simulink model "generic_src"  (Simulink 10.3)
settings: Solver=ode45  StartTime=0.0  StopTime=inf  RelTol=1e-3  EnableMultiTasking=on
undefined symbols (not defined in the file or in its folder): Area_Front, Area_Rear, ay_max_off, ay_max_on, ay_per_mu_max_off, ay_per_mu_max_on, Brake_ratio, brake_valve_ctrl_kP, cat1mode1_higher, cat1mode1_lower, cat1mode2_higher, cat1mode2_lower, cat1mode3_higher, cat1mode3_lower, cat2mode1_higher, cat2mode1_lower, cat2mode2_higher, cat2mode2_lower, cat2mode3_higher, cat2mode3_lower, delta_vel, diff_lock_fac, diff_lock_off, diff_lock_on, ESP_ctrl_kD, ESP_ctrl_kI, ESP_ctrl_kP, ESP_ctrl_restore_kI, ESP_min_throttle_fac, f_ax, f_slip, g, higherlimit_highvel, higherlimit_lowvel, highervel_fac, highervelocity_fac, InitialConditionForIntegrator, limit_acc, limit_selectlow, limit_starting, limit_vdiff, locktime_throttle, lowerlimit_highvel, lowerlimit_lowvel, lowervel_fac, lowervelocity_fac, min_throttle, MPS2KMPH, MSR_ctrl_kD, MSR_ctrl_kI, MSR_ctrl_kP, MSR_min_throttle_fac, PID_kP_sideslip, PID_kP_yawrate, RADpS2RpM, rBrake, RpM2RADpS, SH_SL_switch, sideslip_vel_corr, sidesplip_deviation_max ... (+35)
libraries: CarMaker4SL x136, simulink x55, simulink_extras x6
(part 4 of 9)

== system generic_src/CarMaker/IPG Vehicle/CarAndTrailer/Forces/Tires/TireFR ==
  note: Insert your tire model here.
  Sync_In : Inport
  Load : Inport  Port=2
  vxtrans : Inport  Port=3
  vytrans : Inport  Port=4
  Rim_rotv : Inport  Port=5
  Rim_turnv : Inport  Port=6
  InclinAngle : Inport  Port=7
  muRoad : Inport  Port=8
  Ground{1..11} (11 alike) : Ground
  Terminator{,1..6,12} (8 alike) : Terminator
  Slp : Outport  VectorParamsAs1DForOutWhenUnconnected=off
  Alpha : Outport  Port=2  VectorParamsAs1DForOutWhenUnconnected=off
  TurnSlp : Outport  Port=3  VectorParamsAs1DForOutWhenUnconnected=off
  rBelt_eff : Outport  Port=4  VectorParamsAs1DForOutWhenUnconnected=off
  vBelt : Outport  Port=5  VectorParamsAs1DForOutWhenUnconnected=off
  LongFrc : Outport  Port=6  VectorParamsAs1DForOutWhenUnconnected=off
  SideFrc : Outport  Port=7  VectorParamsAs1DForOutWhenUnconnected=off
  LoadFrc : Outport  Port=8  VectorParamsAs1DForOutWhenUnconnected=off
  OverturnTrq : Outport  Port=9  VectorParamsAs1DForOutWhenUnconnected=off
  RollResist : Outport  Port=10  VectorParamsAs1DForOutWhenUnconnected=off
  AlignTrq : Outport  Port=11  VectorParamsAs1DForOutWhenUnconnected=off
  wires:
  Ground11/1 -> vBelt/1
  Ground10/1 -> rBelt_eff/1
  Ground9/1 -> TurnSlp/1
  Rim_turnv/1 -> Terminator6/1
  Sync_In/1 -> Terminator12/1
  Ground2/1 -> Alpha/1
  Ground3/1 -> LongFrc/1
  Ground4/1 -> SideFrc/1
  Ground5/1 -> OverturnTrq/1
  vxtrans/1 -> Terminator1/1
  vytrans/1 -> Terminator2/1
  Rim_rotv/1 -> Terminator3/1
  InclinAngle/1 -> Terminator4/1
  muRoad/1 -> Terminator5/1
  Load/1 -> Terminator/1
  Ground1/1 -> Slp/1
  Ground6/1 -> LoadFrc/1
  Ground7/1 -> RollResist/1
  Ground8/1 -> AlignTrq/1

== system generic_src/CarMaker/IPG Vehicle/CarAndTrailer/Forces/Tires/TireRL ==
  note: Insert your tire model here.
  Sync_In : Inport
  Load : Inport  Port=2
  vxtrans : Inport  Port=3
  vytrans : Inport  Port=4
  Rim_rotv : Inport  Port=5
  Rim_turnv : Inport  Port=6
  InclinAngle : Inport  Port=7
  muRoad : Inport  Port=8
  Ground{1..11} (11 alike) : Ground
  Terminator{,1..6,12} (8 alike) : Terminator
  Slp : Outport  VectorParamsAs1DForOutWhenUnconnected=off
  Alpha : Outport  Port=2  VectorParamsAs1DForOutWhenUnconnected=off
  TurnSlp : Outport  Port=3  VectorParamsAs1DForOutWhenUnconnected=off
  rBelt_eff : Outport  Port=4  VectorParamsAs1DForOutWhenUnconnected=off
  vBelt : Outport  Port=5  VectorParamsAs1DForOutWhenUnconnected=off
  LongFrc : Outport  Port=6  VectorParamsAs1DForOutWhenUnconnected=off
  SideFrc : Outport  Port=7  VectorParamsAs1DForOutWhenUnconnected=off
  LoadFrc : Outport  Port=8  VectorParamsAs1DForOutWhenUnconnected=off
  OverturnTrq : Outport  Port=9  VectorParamsAs1DForOutWhenUnconnected=off
  RollResist : Outport  Port=10  VectorParamsAs1DForOutWhenUnconnected=off
  AlignTrq : Outport  Port=11  VectorParamsAs1DForOutWhenUnconnected=off
  wires:
  Ground11/1 -> vBelt/1
  Ground10/1 -> rBelt_eff/1
  Ground9/1 -> TurnSlp/1
  Rim_turnv/1 -> Terminator6/1
  Sync_In/1 -> Terminator12/1
  Ground2/1 -> Alpha/1
  Ground3/1 -> LongFrc/1
  Ground4/1 -> SideFrc/1
  Ground5/1 -> OverturnTrq/1
  vxtrans/1 -> Terminator1/1
  vytrans/1 -> Terminator2/1
  Rim_rotv/1 -> Terminator3/1
  InclinAngle/1 -> Terminator4/1
  muRoad/1 -> Terminator5/1
  Load/1 -> Terminator/1
  Ground1/1 -> Slp/1
  Ground6/1 -> LoadFrc/1
  Ground7/1 -> RollResist/1
  Ground8/1 -> AlignTrq/1

== system generic_src/CarMaker/IPG Vehicle/CarAndTrailer/Forces/Tires/TireRR ==
  note: Insert your tire model here.
  Sync_In : Inport
  Load : Inport  Port=2
  vxtrans : Inport  Port=3
  vytrans : Inport  Port=4
  Rim_rotv : Inport  Port=5
  Rim_turnv : Inport  Port=6
  InclinAngle : Inport  Port=7
  muRoad : Inport  Port=8
  Ground{1..11} (11 alike) : Ground
  Terminator{,1..6,12} (8 alike) : Terminator
  Slp : Outport  VectorParamsAs1DForOutWhenUnconnected=off
  Alpha : Outport  Port=2  VectorParamsAs1DForOutWhenUnconnected=off
  TurnSlp : Outport  Port=3  VectorParamsAs1DForOutWhenUnconnected=off
  rBelt_eff : Outport  Port=4  VectorParamsAs1DForOutWhenUnconnected=off
  vBelt : Outport  Port=5  VectorParamsAs1DForOutWhenUnconnected=off
  LongFrc : Outport  Port=6  VectorParamsAs1DForOutWhenUnconnected=off
  SideFrc : Outport  Port=7  VectorParamsAs1DForOutWhenUnconnected=off
  LoadFrc : Outport  Port=8  VectorParamsAs1DForOutWhenUnconnected=off
  OverturnTrq : Outport  Port=9  VectorParamsAs1DForOutWhenUnconnected=off
  RollResist : Outport  Port=10  VectorParamsAs1DForOutWhenUnconnected=off
  AlignTrq : Outport  Port=11  VectorParamsAs1DForOutWhenUnconnected=off
  wires:
  Ground11/1 -> vBelt/1
  Ground10/1 -> rBelt_eff/1
  Ground9/1 -> TurnSlp/1
  Rim_turnv/1 -> Terminator6/1
  Sync_In/1 -> Terminator12/1
  Ground2/1 -> Alpha/1
  Ground3/1 -> LongFrc/1
  Ground4/1 -> SideFrc/1
  Ground5/1 -> OverturnTrq/1
  vxtrans/1 -> Terminator1/1
  vytrans/1 -> Terminator2/1
  Rim_rotv/1 -> Terminator3/1
  InclinAngle/1 -> Terminator4/1
  muRoad/1 -> Terminator5/1
  Load/1 -> Terminator/1
  Ground1/1 -> Slp/1
  Ground6/1 -> LoadFrc/1
  Ground7/1 -> RollResist/1
  Ground8/1 -> AlignTrq/1

== system generic_src/CarMaker/IPG Vehicle/PowerTrain/MCU Example/MyMotorCU/Enabled Subsystem ==
  rotv : Inport
  Trq_trg : Inport  Port=2
  Load : Inport  Port=3
  rotv_trg : Inport  Port=4
  Ratio : Inport  Port=5
  TrqMot_max table : Inport  Port=6
  TrqGen_max table : Inport  Port=7
  rotv_Mot_max : Inport  Port=8
  rotv_Gen_max : Inport  Port=9
  Enable : EnablePort
  Abs : Abs
  Abs1 : Abs
  Abs2 : Abs
  Bus Selector : BusSelector  OutputSignals=x,z
  Bus Selector1 : BusSelector  OutputSignals=x,z
  Compare To Constant : simulink/Logic and Bit Operations/Compare To Constant  relop===  const=-99999  OutDataTypeStr=uint8  ZeroCross=off
  Constant : Constant  Value=0.0
  Constant1 : Constant  Value=0.0
  Gain : Gain  Gain=-1
  Lookup Table Dynamic : simulink/Lookup Tables/Lookup Table Dynamic  LookUpMeth=Interpolation-Use End Values  OutDataType=float('double')  OutScaling=[]  OutputDataTypeScalingMode=Specify via dialog  OutDataTypeStr=float('double')  DoSatur=off
  Lookup Table Dynamic1 : simulink/Lookup Tables/Lookup Table Dynamic  LookUpMeth=Interpolation-Use End Values  OutDataType=float('double')  OutScaling=[]  OutputDataTypeScalingMode=Specify via dialog  OutDataTypeStr=float('double')  DoSatur=off
  MotMode : Subsystem
  Product : Product  RndMeth=Zero
  Product1 : Product  RndMeth=Zero
  Product2 : Product  RndMeth=Zero
  Saturation : Saturate  UpperLimit=1  LowerLimit=-1
  Switch : Switch  Criteria=u2 ~= 0
  Switch1 : Switch  Criteria=u2 ~= 0
  Switch2 : Switch  Criteria=u2 ~= 0
  if condition : Subsystem
  rotv Copy : InportShadow
  Load out : Outport  VectorParamsAs1DForOutWhenUnconnected=off
  TrqMot_max : Outport  Port=2  VectorParamsAs1DForOutWhenUnconnected=off
  TrqGen_max : Outport  Port=3  VectorParamsAs1DForOutWhenUnconnected=off
  wires:
  rotv Copy/1 -> if condition/2(rotv)
  Bus Selector/2 -> Lookup Table Dynamic/3  "<z>"
  Lookup Table Dynamic/1 -> Product1/2
  Abs2/1 -> Switch/1
  Abs1/1 -> Switch/3
  Product/1 -> Lookup Table Dynamic1/1, Lookup Table Dynamic/1  "rotv"
  rotv_trg/1 -> if condition/1(rotv_trg)
  if condition/1(Boolean) -> Switch2/2
  Switch1/1 -> Switch2/3  "Load"
  Constant1/1 -> Switch2/1
  Switch2/1 -> Load out/1
  Saturation/1 -> Switch1/3
  Constant/1 -> Switch1/1
  Compare To Constant/1 -> Switch1/2
  Load/1 -> Saturation/1, Compare To Constant/1
  Trq_trg/1 -> MotMode/1(Trq_trg)
  MotMode/1(Boolean) -> Switch/2
  Gain/1 -> Product2/2
  Product2/1 -> TrqGen_max/1
  Product1/1 -> TrqMot_max/1
  Switch/1 -> if condition/3(lim_rotv)  "lim_rotv"
  rotv_Mot_max/1 -> Abs2/1
  rotv_Gen_max/1 -> Abs1/1
  Lookup Table Dynamic1/1 -> Gain/1
  Bus Selector1/2 -> Lookup Table Dynamic1/3  "<z>"
  Bus Selector1/1 -> Lookup Table Dynamic1/2  "<x>"
  TrqGen_max table/1 -> Bus Selector1/1
  Bus Selector/1 -> Lookup Table Dynamic/2  "<x>"
  TrqMot_max table/1 -> Bus Selector/1
  Abs/1 -> Product/1
  Ratio/1 -> Product1/1, Product2/1, Product/2
  rotv/1 -> MotMode/2(rotv), Abs/1

== system generic_src/CarMaker/IPG Vehicle/PowerTrain/MCU Example/MyMotorCU/ReturnZero ==
  Enable : EnablePort
  Bus Creator : BusCreator  Inputs=3
  Constant : Constant  Value=0.0
  Constant1 : Constant  Value=0.0
  Constant2 : Constant  Value=0.0
  Signal Conversion : SignalConversion  ConversionOutput=Bus copy  OverrideOpt=off
  ReturnZero : Outport  VectorParamsAs1DForOutWhenUnconnected=off
  wires:
  Signal Conversion/1 -> ReturnZero/1
  Constant2/1 -> Bus Creator/3  "TrqGen_max"
  Constant1/1 -> Bus Creator/2  "TrqMot_max"
  Constant/1 -> Bus Creator/1  "Load"
  Bus Creator/1 -> Signal Conversion/1

== system generic_src/CarMaker/IPG Vehicle/PowerTrain/MCU Example/PTMotorCU_In/CreateBus MCU ISGIn ==
  In : Inport
  BusCreator : BusCreator  Inputs=12
  Demux : Demux  Outputs=12
      settings: DisplayOption=none
  Out : Outport  VectorParamsAs1DForOutWhenUnconnected=off
  wires:
  Demux/6 -> BusCreator/6  "MCU ISGIn PwrElec"
  Demux/4 -> BusCreator/4  "MCU ISGIn rotv"
  Demux/3 -> BusCreator/3  "MCU ISGIn rotv_trg"
  Demux/2 -> BusCreator/2  "MCU ISGIn Trq"
  Demux/8 -> BusCreator/8  "MCU ISGIn Current_d"
  Demux/9 -> BusCreator/9  "MCU ISGIn Current_q"
  In/1 -> Demux/1
  Demux/7 -> BusCreator/7  "MCU ISGIn VoltBatt"
  BusCreator/1 -> Out/1
  Demux/1 -> BusCreator/1  "MCU ISGIn Trq_trg"
  Demux/5 -> BusCreator/5  "MCU ISGIn rot"
  Demux/10 -> BusCreator/10  "MCU ISGIn Current_u"
  Demux/11 -> BusCreator/11  "MCU ISGIn Current_v"
  Demux/12 -> BusCreator/12  "MCU ISGIn Current_w"

== system generic_src/CarMaker/IPG Vehicle/PowerTrain/MCU Example/PTMotorCU_In/CreateBus MCU ISGOut ==
  In : Inport
  BusCreator : BusCreator  Inputs=1
  Demux : Demux  Outputs=1
      settings: DisplayOption=none
  Out : Outport  VectorParamsAs1DForOutWhenUnconnected=off
  wires:
  Demux/1 -> BusCreator/1  "MCU ISGIn Load"
  BusCreator/1 -> Out/1
  In/1 -> Demux/1

== system generic_src/CarMaker/IPG Vehicle/PowerTrain/MCU Example/PTMotorCU_In/CreateBus MCU Ignition ==
  In : Inport
  BusCreator : BusCreator  Inputs=1
  Demux : Demux  Outputs=1
      settings: DisplayOption=none
  Out : Outport  VectorParamsAs1DForOutWhenUnconnected=off
  wires:
  Demux/1 -> BusCreator/1  "MCU Ignition"
  BusCreator/1 -> Out/1
  In/1 -> Demux/1

== system generic_src/CarMaker/IPG Vehicle/PowerTrain/MCU Example/PTMotorCU_In/CreateBus MCU MotorIn0 ==
  In : Inport
  BusCreator1 : BusCreator  Inputs=12
  Demux1 : Demux  Outputs=12
      settings: DisplayOption=none
  Out : Outport  VectorParamsAs1DForOutWhenUnconnected=off
  wires:
  In/1 -> Demux1/1
  Demux1/12 -> BusCreator1/12  "MCU MotorIn0 Current_w"
  Demux1/10 -> BusCreator1/10  "MCU MotorIn0 Current_u"
  Demux1/6 -> BusCreator1/6  "MCU MotorIn0 PwrElec"
  Demux1/7 -> BusCreator1/7  "MCU MotorIn0 VoltBatt"
  Demux1/9 -> BusCreator1/9  "MCU MotorIn0 Current_q"
  Demux1/1 -> BusCreator1/1  "MCU MotorIn0 Trq_trg"
  Demux1/3 -> BusCreator1/3  "MCU MotorIn0 rotv_trg"
  BusCreator1/1 -> Out/1
  Demux1/2 -> BusCreator1/2  "MCU MotorIn0 Trq"
  Demux1/4 -> BusCreator1/4  "MCU MotorIn0 rotv"
  Demux1/11 -> BusCreator1/11  "MCU MotorIn0 Current_v"
  Demux1/8 -> BusCreator1/8  "MCU MotorIn0 Current_d"
  Demux1/5 -> BusCreator1/5  "MCU MotorIn0 rot"

== system generic_src/CarMaker/IPG Vehicle/PowerTrain/MCU Example/PTMotorCU_In/CreateBus MCU MotorIn1 ==
  In : Inport
  BusCreator1 : BusCreator  Inputs=12
  Demux1 : Demux  Outputs=12
      settings: DisplayOption=none
  Out : Outport  VectorParamsAs1DForOutWhenUnconnected=off
  wires:
  Demux1/4 -> BusCreator1/4  "MCU MotorIn1 rotv"
  Demux1/10 -> BusCreator1/10  "MCU MotorIn1 Current_u"
  BusCreator1/1 -> Out/1
  Demux1/7 -> BusCreator1/7  "MCU MotorIn1 VoltBatt"
  Demux1/8 -> BusCreator1/8  "MCU MotorIn1 Current_d"
  Demux1/1 -> BusCreator1/1  "MCU MotorIn1 Trq_trg"
  Demux1/9 -> BusCreator1/9  "MCU MotorIn1 Current_q"
  Demux1/5 -> BusCreator1/5  "MCU MotorIn1 rot"
  In/1 -> Demux1/1
  Demux1/2 -> BusCreator1/2  "MCU MotorIn1 Trq"
  Demux1/3 -> BusCreator1/3  "MCU MotorIn1 rotv_trg"
  Demux1/6 -> BusCreator1/6  "MCU MotorIn1 PwrElec"
  Demux1/12 -> BusCreator1/12  "MCU MotorIn1 Current_w"
  Demux1/11 -> BusCreator1/11  "MCU MotorIn1 Current_v"

== system generic_src/CarMaker/IPG Vehicle/PowerTrain/MCU Example/PTMotorCU_In/CreateBus MCU MotorIn2 ==
  In : Inport
  BusCreator1 : BusCreator  Inputs=12
  Demux1 : Demux  Outputs=12
      settings: DisplayOption=none
  Out : Outport  VectorParamsAs1DForOutWhenUnconnected=off
  wires:
  Demux1/1 -> BusCreator1/1  "MCU MotorIn2 Trq_trg"
  Demux1/5 -> BusCreator1/5  "MCU MotorIn2 rot"
  BusCreator1/1 -> Out/1
  Demux1/9 -> BusCreator1/9  "MCU MotorIn2 Current_q"
  Demux1/3 -> BusCreator1/3  "MCU MotorIn2 rotv_trg"
  Demux1/4 -> BusCreator1/4  "MCU MotorIn2 rotv"
  Demux1/7 -> BusCreator1/7  "MCU MotorIn2 VoltBatt"
  Demux1/12 -> BusCreator1/12  "MCU MotorIn2 Current_w"
  In/1 -> Demux1/1
  Demux1/2 -> BusCreator1/2  "MCU MotorIn2 Trq"
  Demux1/8 -> BusCreator1/8  "MCU MotorIn2 Current_d"
  Demux1/11 -> BusCreator1/11  "MCU MotorIn2 Current_v"
  Demux1/6 -> BusCreator1/6  "MCU MotorIn2 PwrElec"
  Demux1/10 -> BusCreator1/10  "MCU MotorIn2 Current_u"

== system generic_src/CarMaker/IPG Vehicle/PowerTrain/MCU Example/PTMotorCU_In/CreateBus MCU MotorIn3 ==
  In : Inport
  BusCreator1 : BusCreator  Inputs=12
  Demux1 : Demux  Outputs=12
      settings: DisplayOption=none
  Out : Outport  VectorParamsAs1DForOutWhenUnconnected=off
  wires:
  BusCreator1/1 -> Out/1
  Demux1/5 -> BusCreator1/5  "MCU MotorIn3 rot"
  Demux1/7 -> BusCreator1/7  "MCU MotorIn3 VoltBatt"
  Demux1/6 -> BusCreator1/6  "MCU MotorIn3 PwrElec"
  Demux1/8 -> BusCreator1/8  "MCU MotorIn3 Current_d"
  Demux1/9 -> BusCreator1/9  "MCU MotorIn3 Current_q"
  Demux1/11 -> BusCreator1/11  "MCU MotorIn3 Current_v"
  Demux1/1 -> BusCreator1/1  "MCU MotorIn3 Trq_trg"
  Demux1/10 -> BusCreator1/10  "MCU MotorIn3 Current_u"
  Demux1/4 -> BusCreator1/4  "MCU MotorIn3 rotv"
  Demux1/12 -> BusCreator1/12  "MCU MotorIn3 Current_w"
  Demux1/2 -> BusCreator1/2  "MCU MotorIn3 Trq"
  In/1 -> Demux1/1
  Demux1/3 -> BusCreator1/3  "MCU MotorIn3 rotv_trg"

== system generic_src/CarMaker/IPG Vehicle/PowerTrain/MCU Example/PTMotorCU_In/CreateBus MCU MotorOut0 ==
  In : Inport
  BusCreator : BusCreator  Inputs=1
  Demux : Demux  Outputs=1
      settings: DisplayOption=none
  Out : Outport  VectorParamsAs1DForOutWhenUnconnected=off
  wires:
  Demux/1 -> BusCreator/1  "MCU MotorOut0 Load"
  BusCreator/1 -> Out/1
  In/1 -> Demux/1

== system generic_src/CarMaker/IPG Vehicle/PowerTrain/MCU Example/PTMotorCU_In/CreateBus MCU MotorOut1 ==
  In : Inport
  BusCreator : BusCreator  Inputs=1
  Demux : Demux  Outputs=1
      settings: DisplayOption=none
  Out : Outport  VectorParamsAs1DForOutWhenUnconnected=off
  wires:
  Demux/1 -> BusCreator/1  "MCU MotorOut1 Load"
  In/1 -> Demux/1
  BusCreator/1 -> Out/1

== system generic_src/CarMaker/IPG Vehicle/PowerTrain/MCU Example/PTMotorCU_In/CreateBus MCU MotorOut2 ==
  In : Inport
  BusCreator : BusCreator  Inputs=1
  Demux : Demux  Outputs=1
      settings: DisplayOption=none
  Out : Outport  VectorParamsAs1DForOutWhenUnconnected=off
  wires:
  Demux/1 -> BusCreator/1  "MCU MotorOut2 Load"
  BusCreator/1 -> Out/1
  In/1 -> Demux/1

== system generic_src/CarMaker/IPG Vehicle/PowerTrain/MCU Example/PTMotorCU_In/CreateBus MCU MotorOut3 ==
  In : Inport
  BusCreator : BusCreator  Inputs=1
  Demux : Demux  Outputs=1
      settings: DisplayOption=none
  Out : Outport  VectorParamsAs1DForOutWhenUnconnected=off
  wires:
  Demux/1 -> BusCreator/1  "MCU MotorOut3 Load"
  BusCreator/1 -> Out/1
  In/1 -> Demux/1

== system generic_src/CarMaker/IPG Vehicle/PowerTrain/MCU Example/PTMotorCU_In/CreateBus MCU_Cfg ISG ==
  In : Inport
  BusCreator : BusCreator  Inputs=8
  Demux : Demux  Outputs=8
      settings: DisplayOption=none
  Out : Outport  VectorParamsAs1DForOutWhenUnconnected=off
  wires:
  BusCreator/1 -> Out/1
  In/1 -> Demux/1
  Demux/4 -> BusCreator/4  "MCU_Cfg ISG rotv_Gen_max"
  Demux/1 -> BusCreator/1  "MCU_Cfg ISG CtrlMode"
  Demux/2 -> BusCreator/2  "MCU_Cfg ISG Ratio"
  Demux/3 -> BusCreator/3  "MCU_Cfg ISG rotv_Mot_max"
  Demux/5 -> BusCreator/5  "MCU_Cfg ISG nPolePairs"
  Demux/6 -> BusCreator/6  "MCU_Cfg ISG L_d"
  Demux/7 -> BusCreator/7  "MCU_Cfg ISG L_q"
  Demux/8 -> BusCreator/8  "MCU_Cfg ISG Psi_PM"

== system generic_src/CarMaker/IPG Vehicle/PowerTrain/MCU Example/PTMotorCU_In/CreateBus MCU_Cfg Misc ==
  In : Inport
  BusCreator : BusCreator  Inputs=1
  Demux : Demux  Outputs=1
      settings: DisplayOption=none
  Out : Outport  VectorParamsAs1DForOutWhenUnconnected=off
  wires:
  Demux/1 -> BusCreator/1  "MCU_Cfg nMotor"
  BusCreator/1 -> Out/1
  In/1 -> Demux/1

== system generic_src/CarMaker/IPG Vehicle/PowerTrain/MCU Example/PTMotorCU_In/CreateBus MCU_Cfg Motor0 ==
  In : Inport
  BusCreator1 : BusCreator  Inputs=8
  Demux1 : Demux  Outputs=8
      settings: DisplayOption=none
  Out : Outport  VectorParamsAs1DForOutWhenUnconnected=off
  wires:
  Demux1/4 -> BusCreator1/4  "MCU_Cfg Motor0 rotv_Gen_max"
  Demux1/2 -> BusCreator1/2  "MCU_Cfg Motor0 Ratio"
  Demux1/3 -> BusCreator1/3  "MCU_Cfg Motor0 rotv_Mot_max"
  Demux1/1 -> BusCreator1/1  "MCU_Cfg Motor0 CtrlMode"
  In/1 -> Demux1/1
  BusCreator1/1 -> Out/1
  Demux1/5 -> BusCreator1/5  "MCU_Cfg Motor0 nPolePairs"
  Demux1/6 -> BusCreator1/6  "MCU_Cfg Motor0 L_d"
  Demux1/7 -> BusCreator1/7  "MCU_Cfg Motor0 L_q"
  Demux1/8 -> BusCreator1/8  "MCU_Cfg Motor0 Psi_PM"

== system generic_src/CarMaker/IPG Vehicle/PowerTrain/MCU Example/PTMotorCU_In/CreateBus MCU_Cfg Motor1 ==
  In : Inport
  BusCreator : BusCreator  Inputs=8
  Demux : Demux  Outputs=8
      settings: DisplayOption=none
  Out : Outport  VectorParamsAs1DForOutWhenUnconnected=off
  wires:
  Demux/4 -> BusCreator/4  "MCU_Cfg Motor1 rotv_Gen_max"
  Demux/2 -> BusCreator/2  "MCU_Cfg Motor1 Ratio"
  Demux/3 -> BusCreator/3  "MCU_Cfg Motor1 rotv_Mot_max"
  Demux/1 -> BusCreator/1  "MCU_Cfg Motor1 CtrlMode"
  In/1 -> Demux/1
  BusCreator/1 -> Out/1
  Demux/5 -> BusCreator/5  "MCU_Cfg Motor1 nPolePairs"
  Demux/6 -> BusCreator/6  "MCU_Cfg Motor1 L_d"
  Demux/7 -> BusCreator/7  "MCU_Cfg Motor1 L_q"
  Demux/8 -> BusCreator/8  "MCU_Cfg Motor1 Psi_PM"

== system generic_src/CarMaker/IPG Vehicle/PowerTrain/MCU Example/PTMotorCU_In/CreateBus MCU_Cfg Motor2 ==
  In : Inport
  BusCreator : BusCreator  Inputs=8
  Demux : Demux  Outputs=8
      settings: DisplayOption=none
  Out : Outport  VectorParamsAs1DForOutWhenUnconnected=off
  wires:
  Demux/4 -> BusCreator/4  "MCU_Cfg Motor2 rotv_Gen_max"
  Demux/1 -> BusCreator/1  "MCU_Cfg Motor2 CtrlMode"
  Demux/2 -> BusCreator/2  "MCU_Cfg Motor2 Ratio"
  Demux/3 -> BusCreator/3  "MCU_Cfg Motor2 rotv_Mot_max"
  BusCreator/1 -> Out/1
  In/1 -> Demux/1
  Demux/5 -> BusCreator/5  "MCU_Cfg Motor2 nPolePairs"
  Demux/6 -> BusCreator/6  "MCU_Cfg Motor2 L_d"
  Demux/7 -> BusCreator/7  "MCU_Cfg Motor2 L_q"
  Demux/8 -> BusCreator/8  "MCU_Cfg Motor2 Psi_PM"

== system generic_src/CarMaker/IPG Vehicle/PowerTrain/MCU Example/PTMotorCU_In/CreateBus MCU_Cfg Motor3 ==
  In : Inport
  BusCreator : BusCreator  Inputs=8
  Demux : Demux  Outputs=8
      settings: DisplayOption=none
  Out : Outport  VectorParamsAs1DForOutWhenUnconnected=off
  wires:
  Demux/4 -> BusCreator/4  "MCU_Cfg Motor3 rotv_Gen_max"
  Demux/1 -> BusCreator/1  "MCU_Cfg Motor3 CtrlMode"
  Demux/2 -> BusCreator/2  "MCU_Cfg Motor3 Ratio"
  Demux/3 -> BusCreator/3  "MCU_Cfg Motor3 rotv_Mot_max"
  BusCreator/1 -> Out/1
  In/1 -> Demux/1
  Demux/5 -> BusCreator/5  "MCU_Cfg Motor3 nPolePairs"
  Demux/6 -> BusCreator/6  "MCU_Cfg Motor3 L_d"
  Demux/7 -> BusCreator/7  "MCU_Cfg Motor3 L_q"
  Demux/8 -> BusCreator/8  "MCU_Cfg Motor3 Psi_PM"

== system generic_src/CarMaker/IPG Vehicle/PowerTrain/PTControl Example/PTC ClutchOut/CreateBus PTC ClutchOut0 ==
  In : Inport
  BusCreator : BusCreator  Inputs=3
  Demux : Demux  Outputs=3
      settings: DisplayOption=none
  Out : Outport  VectorParamsAs1DForOutWhenUnconnected=off
  wires:
  Demux/3 -> BusCreator/3  "PTC ClutchOut0 Trq_out_trg"
  Demux/2 -> BusCreator/2  "PTC ClutchOut0 rotv_out_trg"
  Demux/1 -> BusCreator/1  "PTC ClutchOut0 Pos"
  BusCreator/1 -> Out/1
  In/1 -> Demux/1

== system generic_src/CarMaker/IPG Vehicle/PowerTrain/PTControl Example/PTC ClutchOut/CreateBus PTC ClutchOut1 ==
  In : Inport
  BusCreator : BusCreator  Inputs=3
  Demux : Demux  Outputs=3
      settings: DisplayOption=none
  Out : Outport  VectorParamsAs1DForOutWhenUnconnected=off
  wires:
  Demux/3 -> BusCreator/3  "PTC ClutchOut1 Trq_out_trg"
  Demux/2 -> BusCreator/2  "PTC ClutchOut1 rotv_out_trg"
  Demux/1 -> BusCreator/1  "PTC ClutchOut1 Pos"
  BusCreator/1 -> Out/1
  In/1 -> Demux/1

== system generic_src/CarMaker/IPG Vehicle/PowerTrain/PTControl Example/PTC ClutchOut/CreateBus PTC ClutchOut10 ==
  In : Inport
  BusCreator : BusCreator  Inputs=3
  Demux : Demux  Outputs=3
      settings: DisplayOption=none
  Out : Outport  VectorParamsAs1DForOutWhenUnconnected=off
  wires:
  Demux/3 -> BusCreator/3  "PTC ClutchOut10 Trq_out_trg"
  Demux/2 -> BusCreator/2  "PTC ClutchOut10 rotv_out_trg"
  Demux/1 -> BusCreator/1  "PTC ClutchOut10 Pos"
  BusCreator/1 -> Out/1
  In/1 -> Demux/1

== system generic_src/CarMaker/IPG Vehicle/PowerTrain/PTControl Example/PTC ClutchOut/CreateBus PTC ClutchOut11 ==
  In : Inport
  BusCreator : BusCreator  Inputs=3
  Demux : Demux  Outputs=3
      settings: DisplayOption=none
  Out : Outport  VectorParamsAs1DForOutWhenUnconnected=off
  wires:
  Demux/3 -> BusCreator/3  "PTC ClutchOut11 Trq_out_trg"
  Demux/2 -> BusCreator/2  "PTC ClutchOut11 rotv_out_trg"
  Demux/1 -> BusCreator/1  "PTC ClutchOut11 Pos"
  BusCreator/1 -> Out/1
  In/1 -> Demux/1

== system generic_src/CarMaker/IPG Vehicle/PowerTrain/PTControl Example/PTC ClutchOut/CreateBus PTC ClutchOut2 ==
  In : Inport
  BusCreator : BusCreator  Inputs=3
  Demux : Demux  Outputs=3
      settings: DisplayOption=none
  Out : Outport  VectorParamsAs1DForOutWhenUnconnected=off
  wires:
  Demux/3 -> BusCreator/3  "PTC ClutchOut2 Trq_out_trg"
  Demux/2 -> BusCreator/2  "PTC ClutchOut2 rotv_out_trg"
  Demux/1 -> BusCreator/1  "PTC ClutchOut2 Pos"
  BusCreator/1 -> Out/1
  In/1 -> Demux/1

== system generic_src/CarMaker/IPG Vehicle/PowerTrain/PTControl Example/PTC ClutchOut/CreateBus PTC ClutchOut3 ==
  In : Inport
  BusCreator : BusCreator  Inputs=3
  Demux : Demux  Outputs=3
      settings: DisplayOption=none
  Out : Outport  VectorParamsAs1DForOutWhenUnconnected=off
  wires:
  Demux/3 -> BusCreator/3  "PTC ClutchOut3 Trq_out_trg"
  Demux/2 -> BusCreator/2  "PTC ClutchOut3 rotv_out_trg"
  Demux/1 -> BusCreator/1  "PTC ClutchOut3 Pos"
  BusCreator/1 -> Out/1
  In/1 -> Demux/1

== system generic_src/CarMaker/IPG Vehicle/PowerTrain/PTControl Example/PTC ClutchOut/CreateBus PTC ClutchOut4 ==
  In : Inport
  BusCreator : BusCreator  Inputs=3
  Demux : Demux  Outputs=3
      settings: DisplayOption=none
  Out : Outport  VectorParamsAs1DForOutWhenUnconnected=off
  wires:
  Demux/3 -> BusCreator/3  "PTC ClutchOut4 Trq_out_trg"
  Demux/2 -> BusCreator/2  "PTC ClutchOut4 rotv_out_trg"
  Demux/1 -> BusCreator/1  "PTC ClutchOut4 Pos"
  BusCreator/1 -> Out/1
  In/1 -> Demux/1

== system generic_src/CarMaker/IPG Vehicle/PowerTrain/PTControl Example/PTC ClutchOut/CreateBus PTC ClutchOut5 ==
  In : Inport
  BusCreator : BusCreator  Inputs=3
  Demux : Demux  Outputs=3
      settings: DisplayOption=none
  Out : Outport  VectorParamsAs1DForOutWhenUnconnected=off
  wires:
  Demux/3 -> BusCreator/3  "PTC ClutchOut5 Trq_out_trg"
  Demux/2 -> BusCreator/2  "PTC ClutchOut5 rotv_out_trg"
  Demux/1 -> BusCreator/1  "PTC ClutchOut5 Pos"
  BusCreator/1 -> Out/1
  In/1 -> Demux/1

== system generic_src/CarMaker/IPG Vehicle/PowerTrain/PTControl Example/PTC ClutchOut/CreateBus PTC ClutchOut6 ==
  In : Inport
  BusCreator : BusCreator  Inputs=3
  Demux : Demux  Outputs=3
      settings: DisplayOption=none
  Out : Outport  VectorParamsAs1DForOutWhenUnconnected=off
  wires:
  Demux/3 -> BusCreator/3  "PTC ClutchOut6 Trq_out_trg"
  Demux/2 -> BusCreator/2  "PTC ClutchOut6 rotv_out_trg"
  Demux/1 -> BusCreator/1  "PTC ClutchOut6 Pos"
  BusCreator/1 -> Out/1
  In/1 -> Demux/1

== system generic_src/CarMaker/IPG Vehicle/PowerTrain/PTControl Example/PTC ClutchOut/CreateBus PTC ClutchOut7 ==
  In : Inport
  BusCreator : BusCreator  Inputs=3
  Demux : Demux  Outputs=3
      settings: DisplayOption=none
  Out : Outport  VectorParamsAs1DForOutWhenUnconnected=off
  wires:
  Demux/3 -> BusCreator/3  "PTC ClutchOut7 Trq_out_trg"
  Demux/2 -> BusCreator/2  "PTC ClutchOut7 rotv_out_trg"
  Demux/1 -> BusCreator/1  "PTC ClutchOut7 Pos"
  BusCreator/1 -> Out/1
  In/1 -> Demux/1

== system generic_src/CarMaker/IPG Vehicle/PowerTrain/PTControl Example/PTC ClutchOut/CreateBus PTC ClutchOut8 ==
  In : Inport
  BusCreator : BusCreator  Inputs=3
  Demux : Demux  Outputs=3
      settings: DisplayOption=none
  Out : Outport  VectorParamsAs1DForOutWhenUnconnected=off
  wires:
  Demux/3 -> BusCreator/3  "PTC ClutchOut8 Trq_out_trg"
  Demux/2 -> BusCreator/2  "PTC ClutchOut8 rotv_out_trg"
  Demux/1 -> BusCreator/1  "PTC ClutchOut8 Pos"
  BusCreator/1 -> Out/1
  In/1 -> Demux/1

== system generic_src/CarMaker/IPG Vehicle/PowerTrain/PTControl Example/PTC ClutchOut/CreateBus PTC ClutchOut9 ==
  In : Inport
  BusCreator : BusCreator  Inputs=3
  Demux : Demux  Outputs=3
      settings: DisplayOption=none
  Out : Outport  VectorParamsAs1DForOutWhenUnconnected=off
  wires:
  Demux/3 -> BusCreator/3  "PTC ClutchOut9 Trq_out_trg"
  Demux/2 -> BusCreator/2  "PTC ClutchOut9 rotv_out_trg"
  Demux/1 -> BusCreator/1  "PTC ClutchOut9 Pos"
  BusCreator/1 -> Out/1
  In/1 -> Demux/1

== system generic_src/CarMaker/IPG Vehicle/PowerTrain/PTControl Example/PTC GearBoxOut/CreateBus PTC GearboxOut0 ==
  In : Inport
  BusCreator : BusCreator  Inputs=12
  Demux : Demux  Outputs=12
      settings: DisplayOption=none
  Out : Outport  VectorParamsAs1DForOutWhenUnconnected=off
  wires:
  Demux/12 -> BusCreator/12  "PTC GearboxOut0 Clutch_dis Trq_out_trg"
  Demux/11 -> BusCreator/11  "PTC GearboxOut0 Clutch_dis rotv_out_trg"
  Demux/10 -> BusCreator/10  "PTC GearboxOut0 Clutch_dis Pos"
  Demux/9 -> BusCreator/9  "PTC GearboxOut0 Clutch Trq_out_trg"
  Demux/8 -> BusCreator/8  "PTC GearboxOut0 Clutch rotv_out_trg"
  Demux/7 -> BusCreator/7  "PTC GearboxOut0 Clutch Pos"
  Demux/6 -> BusCreator/6  "PTC GearboxOut0 Trq_out_trg"
  Demux/5 -> BusCreator/5  "PTC GearboxOut0 rotv_in_trg"
  Demux/4 -> BusCreator/4  "PTC GearboxOut0 i_trg"
  Demux/3 -> BusCreator/3  "PTC GearboxOut0 set_ParkBrake"
  Demux/2 -> BusCreator/2  "PTC GearboxOut0 GearNoTrg_dis"
  Demux/1 -> BusCreator/1  "PTC GearboxOut0 GearNoTrg"
  BusCreator/1 -> Out/1
  In/1 -> Demux/1

== system generic_src/CarMaker/IPG Vehicle/PowerTrain/PTControl Example/PTC GearBoxOut/CreateBus PTC GearboxOut1 ==
  In : Inport
  BusCreator : BusCreator  Inputs=12
  Demux : Demux  Outputs=12
      settings: DisplayOption=none
  Out : Outport  VectorParamsAs1DForOutWhenUnconnected=off
  wires:
  Demux/12 -> BusCreator/12  "PTC GearboxOut1 Clutch_dis Trq_out_trg"
  Demux/11 -> BusCreator/11  "PTC GearboxOut1 Clutch_dis rotv_out_trg"
  Demux/10 -> BusCreator/10  "PTC GearboxOut1 Clutch_dis Pos"
  Demux/9 -> BusCreator/9  "PTC GearboxOut1 Clutch Trq_out_trg"
  Demux/8 -> BusCreator/8  "PTC GearboxOut1 Clutch rotv_out_trg"
  Demux/7 -> BusCreator/7  "PTC GearboxOut1 Clutch Pos"
  Demux/6 -> BusCreator/6  "PTC GearboxOut1 Trq_out_trg"
  Demux/5 -> BusCreator/5  "PTC GearboxOut1 rotv_in_trg"
  Demux/4 -> BusCreator/4  "PTC GearboxOut1 i_trg"
  Demux/3 -> BusCreator/3  "PTC GearboxOut1 set_ParkBrake"
  Demux/2 -> BusCreator/2  "PTC GearboxOut1 GearNoTrg_dis"
  Demux/1 -> BusCreator/1  "PTC GearboxOut1 GearNoTrg"
  BusCreator/1 -> Out/1
  In/1 -> Demux/1

== system generic_src/CarMaker/IPG Vehicle/PowerTrain/PTControl Example/PTC GearBoxOut/CreateBus PTC GearboxOut10 ==
  In : Inport
  BusCreator : BusCreator  Inputs=12
  Demux : Demux  Outputs=12
      settings: DisplayOption=none
  Out : Outport  VectorParamsAs1DForOutWhenUnconnected=off
  wires:
  Demux/12 -> BusCreator/12  "PTC GearboxOut10 Clutch_dis Trq_out_trg"
  Demux/11 -> BusCreator/11  "PTC GearboxOut10 Clutch_dis rotv_out_trg"
  Demux/10 -> BusCreator/10  "PTC GearboxOut10 Clutch_dis Pos"
  Demux/9 -> BusCreator/9  "PTC GearboxOut10 Clutch Trq_out_trg"
  Demux/8 -> BusCreator/8  "PTC GearboxOut10 Clutch rotv_out_trg"
  Demux/7 -> BusCreator/7  "PTC GearboxOut10 Clutch Pos"
  Demux/6 -> BusCreator/6  "PTC GearboxOut10 Trq_out_trg"
  Demux/5 -> BusCreator/5  "PTC GearboxOut10 rotv_in_trg"
  Demux/4 -> BusCreator/4  "PTC GearboxOut10 i_trg"
  Demux/3 -> BusCreator/3  "PTC GearboxOut10 set_ParkBrake"
  Demux/2 -> BusCreator/2  "PTC GearboxOut10 GearNoTrg_dis"
  Demux/1 -> BusCreator/1  "PTC GearboxOut10 GearNoTrg"
  BusCreator/1 -> Out/1
  In/1 -> Demux/1

== system generic_src/CarMaker/IPG Vehicle/PowerTrain/PTControl Example/PTC GearBoxOut/CreateBus PTC GearboxOut11 ==
  In : Inport
  BusCreator : BusCreator  Inputs=12
  Demux : Demux  Outputs=12
      settings: DisplayOption=none
  Out : Outport  VectorParamsAs1DForOutWhenUnconnected=off
  wires:
  Demux/12 -> BusCreator/12  "PTC GearboxOut11 Clutch_dis Trq_out_trg"
  Demux/11 -> BusCreator/11  "PTC GearboxOut11 Clutch_dis rotv_out_trg"
  Demux/10 -> BusCreator/10  "PTC GearboxOut11 Clutch_dis Pos"
  Demux/9 -> BusCreator/9  "PTC GearboxOut11 Clutch Trq_out_trg"
  Demux/8 -> BusCreator/8  "PTC GearboxOut11 Clutch rotv_out_trg"
  Demux/7 -> BusCreator/7  "PTC GearboxOut11 Clutch Pos"
  Demux/6 -> BusCreator/6  "PTC GearboxOut11 Trq_out_trg"
  Demux/5 -> BusCreator/5  "PTC GearboxOut11 rotv_in_trg"
  Demux/4 -> BusCreator/4  "PTC GearboxOut11 i_trg"
  Demux/3 -> BusCreator/3  "PTC GearboxOut11 set_ParkBrake"
  Demux/2 -> BusCreator/2  "PTC GearboxOut11 GearNoTrg_dis"
  Demux/1 -> BusCreator/1  "PTC GearboxOut11 GearNoTrg"
  BusCreator/1 -> Out/1
  In/1 -> Demux/1

== system generic_src/CarMaker/IPG Vehicle/PowerTrain/PTControl Example/PTC GearBoxOut/CreateBus PTC GearboxOut2 ==
  In : Inport
  BusCreator : BusCreator  Inputs=12
  Demux : Demux  Outputs=12
      settings: DisplayOption=none
  Out : Outport  VectorParamsAs1DForOutWhenUnconnected=off
  wires:
  Demux/12 -> BusCreator/12  "PTC GearboxOut2 Clutch_dis Trq_out_trg"
  Demux/11 -> BusCreator/11  "PTC GearboxOut2 Clutch_dis rotv_out_trg"
  Demux/10 -> BusCreator/10  "PTC GearboxOut2 Clutch_dis Pos"
  Demux/9 -> BusCreator/9  "PTC GearboxOut2 Clutch Trq_out_trg"
  Demux/8 -> BusCreator/8  "PTC GearboxOut2 Clutch rotv_out_trg"
  Demux/7 -> BusCreator/7  "PTC GearboxOut2 Clutch Pos"
  Demux/6 -> BusCreator/6  "PTC GearboxOut2 Trq_out_trg"
  Demux/5 -> BusCreator/5  "PTC GearboxOut2 rotv_in_trg"
  Demux/4 -> BusCreator/4  "PTC GearboxOut2 i_trg"
  Demux/3 -> BusCreator/3  "PTC GearboxOut2 set_ParkBrake"
  Demux/2 -> BusCreator/2  "PTC GearboxOut2 GearNoTrg_dis"
  Demux/1 -> BusCreator/1  "PTC GearboxOut2 GearNoTrg"
  BusCreator/1 -> Out/1
  In/1 -> Demux/1

== system generic_src/CarMaker/IPG Vehicle/PowerTrain/PTControl Example/PTC GearBoxOut/CreateBus PTC GearboxOut3 ==
  In : Inport
  BusCreator : BusCreator  Inputs=12
  Demux : Demux  Outputs=12
      settings: DisplayOption=none
  Out : Outport  VectorParamsAs1DForOutWhenUnconnected=off
  wires:
  Demux/12 -> BusCreator/12  "PTC GearboxOut3 Clutch_dis Trq_out_trg"
  Demux/11 -> BusCreator/11  "PTC GearboxOut3 Clutch_dis rotv_out_trg"
  Demux/10 -> BusCreator/10  "PTC GearboxOut3 Clutch_dis Pos"
  Demux/9 -> BusCreator/9  "PTC GearboxOut3 Clutch Trq_out_trg"
  Demux/8 -> BusCreator/8  "PTC GearboxOut3 Clutch rotv_out_trg"
  Demux/7 -> BusCreator/7  "PTC GearboxOut3 Clutch Pos"
  Demux/6 -> BusCreator/6  "PTC GearboxOut3 Trq_out_trg"
  Demux/5 -> BusCreator/5  "PTC GearboxOut3 rotv_in_trg"
  Demux/4 -> BusCreator/4  "PTC GearboxOut3 i_trg"
  Demux/3 -> BusCreator/3  "PTC GearboxOut3 set_ParkBrake"
  Demux/2 -> BusCreator/2  "PTC GearboxOut3 GearNoTrg_dis"
  Demux/1 -> BusCreator/1  "PTC GearboxOut3 GearNoTrg"
  BusCreator/1 -> Out/1
  In/1 -> Demux/1

== system generic_src/CarMaker/IPG Vehicle/PowerTrain/PTControl Example/PTC GearBoxOut/CreateBus PTC GearboxOut4 ==
  In : Inport
  BusCreator : BusCreator  Inputs=12
  Demux : Demux  Outputs=12
      settings: DisplayOption=none
  Out : Outport  VectorParamsAs1DForOutWhenUnconnected=off
  wires:
  Demux/12 -> BusCreator/12  "PTC GearboxOut4 Clutch_dis Trq_out_trg"
  Demux/11 -> BusCreator/11  "PTC GearboxOut4 Clutch_dis rotv_out_trg"
  Demux/10 -> BusCreator/10  "PTC GearboxOut4 Clutch_dis Pos"
  Demux/9 -> BusCreator/9  "PTC GearboxOut4 Clutch Trq_out_trg"
  Demux/8 -> BusCreator/8  "PTC GearboxOut4 Clutch rotv_out_trg"
  Demux/7 -> BusCreator/7  "PTC GearboxOut4 Clutch Pos"
  Demux/6 -> BusCreator/6  "PTC GearboxOut4 Trq_out_trg"
  Demux/5 -> BusCreator/5  "PTC GearboxOut4 rotv_in_trg"
  Demux/4 -> BusCreator/4  "PTC GearboxOut4 i_trg"
  Demux/3 -> BusCreator/3  "PTC GearboxOut4 set_ParkBrake"
  Demux/2 -> BusCreator/2  "PTC GearboxOut4 GearNoTrg_dis"
  Demux/1 -> BusCreator/1  "PTC GearboxOut4 GearNoTrg"
  BusCreator/1 -> Out/1
  In/1 -> Demux/1

== system generic_src/CarMaker/IPG Vehicle/PowerTrain/PTControl Example/PTC GearBoxOut/CreateBus PTC GearboxOut5 ==
  In : Inport
  BusCreator : BusCreator  Inputs=12
  Demux : Demux  Outputs=12
      settings: DisplayOption=none
  Out : Outport  VectorParamsAs1DForOutWhenUnconnected=off
  wires:
  Demux/12 -> BusCreator/12  "PTC GearboxOut5 Clutch_dis Trq_out_trg"
  Demux/11 -> BusCreator/11  "PTC GearboxOut5 Clutch_dis rotv_out_trg"
  Demux/10 -> BusCreator/10  "PTC GearboxOut5 Clutch_dis Pos"
  Demux/9 -> BusCreator/9  "PTC GearboxOut5 Clutch Trq_out_trg"
  Demux/8 -> BusCreator/8  "PTC GearboxOut5 Clutch rotv_out_trg"
  Demux/7 -> BusCreator/7  "PTC GearboxOut5 Clutch Pos"
  Demux/6 -> BusCreator/6  "PTC GearboxOut5 Trq_out_trg"
  Demux/5 -> BusCreator/5  "PTC GearboxOut5 rotv_in_trg"
  Demux/4 -> BusCreator/4  "PTC GearboxOut5 i_trg"
  Demux/3 -> BusCreator/3  "PTC GearboxOut5 set_ParkBrake"
  Demux/2 -> BusCreator/2  "PTC GearboxOut5 GearNoTrg_dis"
  Demux/1 -> BusCreator/1  "PTC GearboxOut5 GearNoTrg"
  BusCreator/1 -> Out/1
  In/1 -> Demux/1

== system generic_src/CarMaker/IPG Vehicle/PowerTrain/PTControl Example/PTC GearBoxOut/CreateBus PTC GearboxOut6 ==
  In : Inport
  BusCreator : BusCreator  Inputs=12
  Demux : Demux  Outputs=12
      settings: DisplayOption=none
  Out : Outport  VectorParamsAs1DForOutWhenUnconnected=off
  wires:
  Demux/12 -> BusCreator/12  "PTC GearboxOut6 Clutch_dis Trq_out_trg"
  Demux/11 -> BusCreator/11  "PTC GearboxOut6 Clutch_dis rotv_out_trg"
  Demux/10 -> BusCreator/10  "PTC GearboxOut6 Clutch_dis Pos"
  Demux/9 -> BusCreator/9  "PTC GearboxOut6 Clutch Trq_out_trg"
  Demux/8 -> BusCreator/8  "PTC GearboxOut6 Clutch rotv_out_trg"
  Demux/7 -> BusCreator/7  "PTC GearboxOut6 Clutch Pos"
  Demux/6 -> BusCreator/6  "PTC GearboxOut6 Trq_out_trg"
  Demux/5 -> BusCreator/5  "PTC GearboxOut6 rotv_in_trg"
  Demux/4 -> BusCreator/4  "PTC GearboxOut6 i_trg"
  Demux/3 -> BusCreator/3  "PTC GearboxOut6 set_ParkBrake"
  Demux/2 -> BusCreator/2  "PTC GearboxOut6 GearNoTrg_dis"
  Demux/1 -> BusCreator/1  "PTC GearboxOut6 GearNoTrg"
  BusCreator/1 -> Out/1
  In/1 -> Demux/1

== system generic_src/CarMaker/IPG Vehicle/PowerTrain/PTControl Example/PTC GearBoxOut/CreateBus PTC GearboxOut7 ==
  In : Inport
  BusCreator : BusCreator  Inputs=12
  Demux : Demux  Outputs=12
      settings: DisplayOption=none
  Out : Outport  VectorParamsAs1DForOutWhenUnconnected=off
  wires:
  Demux/12 -> BusCreator/12  "PTC GearboxOut7 Clutch_dis Trq_out_trg"
  Demux/11 -> BusCreator/11  "PTC GearboxOut7 Clutch_dis rotv_out_trg"
  Demux/10 -> BusCreator/10  "PTC GearboxOut7 Clutch_dis Pos"
  Demux/9 -> BusCreator/9  "PTC GearboxOut7 Clutch Trq_out_trg"
  Demux/8 -> BusCreator/8  "PTC GearboxOut7 Clutch rotv_out_trg"
  Demux/7 -> BusCreator/7  "PTC GearboxOut7 Clutch Pos"
  Demux/6 -> BusCreator/6  "PTC GearboxOut7 Trq_out_trg"
  Demux/5 -> BusCreator/5  "PTC GearboxOut7 rotv_in_trg"
  Demux/4 -> BusCreator/4  "PTC GearboxOut7 i_trg"
  Demux/3 -> BusCreator/3  "PTC GearboxOut7 set_ParkBrake"
  Demux/2 -> BusCreator/2  "PTC GearboxOut7 GearNoTrg_dis"
  Demux/1 -> BusCreator/1  "PTC GearboxOut7 GearNoTrg"
  BusCreator/1 -> Out/1
  In/1 -> Demux/1

== system generic_src/CarMaker/IPG Vehicle/PowerTrain/PTControl Example/PTC GearBoxOut/CreateBus PTC GearboxOut8 ==
  In : Inport
  BusCreator : BusCreator  Inputs=12
  Demux : Demux  Outputs=12
      settings: DisplayOption=none
  Out : Outport  VectorParamsAs1DForOutWhenUnconnected=off
  wires:
  Demux/12 -> BusCreator/12  "PTC GearboxOut8 Clutch_dis Trq_out_trg"
  Demux/11 -> BusCreator/11  "PTC GearboxOut8 Clutch_dis rotv_out_trg"
  Demux/10 -> BusCreator/10  "PTC GearboxOut8 Clutch_dis Pos"
  Demux/9 -> BusCreator/9  "PTC GearboxOut8 Clutch Trq_out_trg"
  Demux/8 -> BusCreator/8  "PTC GearboxOut8 Clutch rotv_out_trg"
  Demux/7 -> BusCreator/7  "PTC GearboxOut8 Clutch Pos"
  Demux/6 -> BusCreator/6  "PTC GearboxOut8 Trq_out_trg"
  Demux/5 -> BusCreator/5  "PTC GearboxOut8 rotv_in_trg"
  Demux/4 -> BusCreator/4  "PTC GearboxOut8 i_trg"
  Demux/3 -> BusCreator/3  "PTC GearboxOut8 set_ParkBrake"
  Demux/2 -> BusCreator/2  "PTC GearboxOut8 GearNoTrg_dis"
  Demux/1 -> BusCreator/1  "PTC GearboxOut8 GearNoTrg"
  BusCreator/1 -> Out/1
  In/1 -> Demux/1

== system generic_src/CarMaker/IPG Vehicle/PowerTrain/PTControl Example/PTC GearBoxOut/CreateBus PTC GearboxOut9 ==
  In : Inport
  BusCreator : BusCreator  Inputs=12
  Demux : Demux  Outputs=12
      settings: DisplayOption=none
  Out : Outport  VectorParamsAs1DForOutWhenUnconnected=off
  wires:
  Demux/12 -> BusCreator/12  "PTC GearboxOut9 Clutch_dis Trq_out_trg"
  Demux/11 -> BusCreator/11  "PTC GearboxOut9 Clutch_dis rotv_out_trg"
  Demux/10 -> BusCreator/10  "PTC GearboxOut9 Clutch_dis Pos"
  Demux/9 -> BusCreator/9  "PTC GearboxOut9 Clutch Trq_out_trg"
  Demux/8 -> BusCreator/8  "PTC GearboxOut9 Clutch rotv_out_trg"
  Demux/7 -> BusCreator/7  "PTC GearboxOut9 Clutch Pos"
  Demux/6 -> BusCreator/6  "PTC GearboxOut9 Trq_out_trg"
  Demux/5 -> BusCreator/5  "PTC GearboxOut9 rotv_in_trg"
  Demux/4 -> BusCreator/4  "PTC GearboxOut9 i_trg"
  Demux/3 -> BusCreator/3  "PTC GearboxOut9 set_ParkBrake"
  Demux/2 -> BusCreator/2  "PTC GearboxOut9 GearNoTrg_dis"
  Demux/1 -> BusCreator/1  "PTC GearboxOut9 GearNoTrg"
  BusCreator/1 -> Out/1
  In/1 -> Demux/1

== system generic_src/CarMaker/IPG Vehicle/PowerTrain/PTControl Example/PTC MotorOut/CreateBus PTC MotorOut0 ==
  In : Inport
  BusCreator : BusCreator  Inputs=3
  Demux : Demux  Outputs=3
      settings: DisplayOption=none
  Out : Outport  VectorParamsAs1DForOutWhenUnconnected=off
  wires:
  Demux/3 -> BusCreator/3  "PTC MotorOut0 rotv_trg"
  Demux/2 -> BusCreator/2  "PTC MotorOut0 Trq_trg"
  Demux/1 -> BusCreator/1  "PTC MotorOut0 Load"
  BusCreator/1 -> Out/1
  In/1 -> Demux/1

== system generic_src/CarMaker/IPG Vehicle/PowerTrain/PTControl Example/PTC MotorOut/CreateBus PTC MotorOut1 ==
  In : Inport
  BusCreator : BusCreator  Inputs=3
  Demux : Demux  Outputs=3
      settings: DisplayOption=none
  Out : Outport  VectorParamsAs1DForOutWhenUnconnected=off
  wires:
  Demux/3 -> BusCreator/3  "PTC MotorOut1 rotv_trg"
  Demux/2 -> BusCreator/2  "PTC MotorOut1 Trq_trg"
  Demux/1 -> BusCreator/1  "PTC MotorOut1 Load"
  BusCreator/1 -> Out/1
  In/1 -> Demux/1

== system generic_src/CarMaker/IPG Vehicle/PowerTrain/PTControl Example/PTC MotorOut/CreateBus PTC MotorOut10 ==
  In : Inport
  BusCreator : BusCreator  Inputs=3
  Demux : Demux  Outputs=3
      settings: DisplayOption=none
  Out : Outport  VectorParamsAs1DForOutWhenUnconnected=off
  wires:
  Demux/3 -> BusCreator/3  "PTC MotorOut10 rotv_trg"
  Demux/2 -> BusCreator/2  "PTC MotorOut10 Trq_trg"
  Demux/1 -> BusCreator/1  "PTC MotorOut10 Load"
  BusCreator/1 -> Out/1
  In/1 -> Demux/1

== system generic_src/CarMaker/IPG Vehicle/PowerTrain/PTControl Example/PTC MotorOut/CreateBus PTC MotorOut11 ==
  In : Inport
  BusCreator : BusCreator  Inputs=3
  Demux : Demux  Outputs=3
      settings: DisplayOption=none
  Out : Outport  VectorParamsAs1DForOutWhenUnconnected=off
  wires:
  Demux/3 -> BusCreator/3  "PTC MotorOut11 rotv_trg"
  Demux/2 -> BusCreator/2  "PTC MotorOut11 Trq_trg"
  Demux/1 -> BusCreator/1  "PTC MotorOut11 Load"
  BusCreator/1 -> Out/1
  In/1 -> Demux/1

== system generic_src/CarMaker/IPG Vehicle/PowerTrain/PTControl Example/PTC MotorOut/CreateBus PTC MotorOut2 ==
  In : Inport
  BusCreator : BusCreator  Inputs=3
  Demux : Demux  Outputs=3
      settings: DisplayOption=none
  Out : Outport  VectorParamsAs1DForOutWhenUnconnected=off
  wires:
  Demux/3 -> BusCreator/3  "PTC MotorOut2 rotv_trg"
  Demux/2 -> BusCreator/2  "PTC MotorOut2 Trq_trg"
  Demux/1 -> BusCreator/1  "PTC MotorOut2 Load"
  BusCreator/1 -> Out/1
  In/1 -> Demux/1

== system generic_src/CarMaker/IPG Vehicle/PowerTrain/PTControl Example/PTC MotorOut/CreateBus PTC MotorOut3 ==
  In : Inport
  BusCreator : BusCreator  Inputs=3
  Demux : Demux  Outputs=3
      settings: DisplayOption=none
  Out : Outport  VectorParamsAs1DForOutWhenUnconnected=off
  wires:
  Demux/3 -> BusCreator/3  "PTC MotorOut3 rotv_trg"
  Demux/2 -> BusCreator/2  "PTC MotorOut3 Trq_trg"
  Demux/1 -> BusCreator/1  "PTC MotorOut3 Load"
  BusCreator/1 -> Out/1
  In/1 -> Demux/1

== system generic_src/CarMaker/IPG Vehicle/PowerTrain/PTControl Example/PTC MotorOut/CreateBus PTC MotorOut4 ==
  In : Inport
  BusCreator : BusCreator  Inputs=3
  Demux : Demux  Outputs=3
      settings: DisplayOption=none
  Out : Outport  VectorParamsAs1DForOutWhenUnconnected=off
  wires:
  Demux/3 -> BusCreator/3  "PTC MotorOut4 rotv_trg"
  Demux/2 -> BusCreator/2  "PTC MotorOut4 Trq_trg"
  Demux/1 -> BusCreator/1  "PTC MotorOut4 Load"
  BusCreator/1 -> Out/1
  In/1 -> Demux/1

== system generic_src/CarMaker/IPG Vehicle/PowerTrain/PTControl Example/PTC MotorOut/CreateBus PTC MotorOut5 ==
  In : Inport
  BusCreator : BusCreator  Inputs=3
  Demux : Demux  Outputs=3
      settings: DisplayOption=none
  Out : Outport  VectorParamsAs1DForOutWhenUnconnected=off
  wires:
  Demux/3 -> BusCreator/3  "PTC MotorOut5 rotv_trg"
  Demux/2 -> BusCreator/2  "PTC MotorOut5 Trq_trg"
  Demux/1 -> BusCreator/1  "PTC MotorOut5 Load"
  BusCreator/1 -> Out/1
  In/1 -> Demux/1

== system generic_src/CarMaker/IPG Vehicle/PowerTrain/PTControl Example/PTC MotorOut/CreateBus PTC MotorOut6 ==
  In : Inport
  BusCreator : BusCreator  Inputs=3
  Demux : Demux  Outputs=3
      settings: DisplayOption=none
  Out : Outport  VectorParamsAs1DForOutWhenUnconnected=off
  wires:
  Demux/3 -> BusCreator/3  "PTC MotorOut6 rotv_trg"
  Demux/2 -> BusCreator/2  "PTC MotorOut6 Trq_trg"
  Demux/1 -> BusCreator/1  "PTC MotorOut6 Load"
  BusCreator/1 -> Out/1
  In/1 -> Demux/1

== system generic_src/CarMaker/IPG Vehicle/PowerTrain/PTControl Example/PTC MotorOut/CreateBus PTC MotorOut7 ==
  In : Inport
  BusCreator : BusCreator  Inputs=3
  Demux : Demux  Outputs=3
      settings: DisplayOption=none
  Out : Outport  VectorParamsAs1DForOutWhenUnconnected=off
  wires:
  Demux/3 -> BusCreator/3  "PTC MotorOut7 rotv_trg"
  Demux/2 -> BusCreator/2  "PTC MotorOut7 Trq_trg"
  Demux/1 -> BusCreator/1  "PTC MotorOut7 Load"
  BusCreator/1 -> Out/1
  In/1 -> Demux/1

== system generic_src/CarMaker/IPG Vehicle/PowerTrain/PTControl Example/PTC MotorOut/CreateBus PTC MotorOut8 ==
  In : Inport
  BusCreator : BusCreator  Inputs=3
  Demux : Demux  Outputs=3
      settings: DisplayOption=none
  Out : Outport  VectorParamsAs1DForOutWhenUnconnected=off
  wires:
  Demux/3 -> BusCreator/3  "PTC MotorOut8 rotv_trg"
  Demux/2 -> BusCreator/2  "PTC MotorOut8 Trq_trg"
  Demux/1 -> BusCreator/1  "PTC MotorOut8 Load"
  BusCreator/1 -> Out/1
  In/1 -> Demux/1

== system generic_src/CarMaker/IPG Vehicle/PowerTrain/PTControl Example/PTC MotorOut/CreateBus PTC MotorOut9 ==
  In : Inport
  BusCreator : BusCreator  Inputs=3
  Demux : Demux  Outputs=3
      settings: DisplayOption=none
  Out : Outport  VectorParamsAs1DForOutWhenUnconnected=off
  wires:
  Demux/3 -> BusCreator/3  "PTC MotorOut9 rotv_trg"
  Demux/2 -> BusCreator/2  "PTC MotorOut9 Trq_trg"
  Demux/1 -> BusCreator/1  "PTC MotorOut9 Load"
  BusCreator/1 -> Out/1
  In/1 -> Demux/1

== system generic_src/CarMaker/IPG Vehicle/PowerTrain/PTControl Example/PTControl Example/Engine ==
  Gas : Inport
  Engine_on : Inport  Port=2
  Constant : Constant
  Constant1 : Constant  Value=0
  Constant3 : Constant  Value=0
  Mux : Mux  Inputs=5
  NOTSET0 : Constant  Value=-99999
  NOTSET1 : Constant  Value=-99999
  NOTSET2 : Constant  Value=-99999
  Switch : Switch  Criteria=u2 ~= 0
  Switch1 : Switch  Criteria=u2 ~= 0
  EngineOut : Outport  VectorParamsAs1DForOutWhenUnconnected=off
  wires:
  Constant/1 -> Switch/1
  Mux/1 -> EngineOut/1
  Constant1/1 -> Switch/3
  Engine_on/1 -> Switch/2, Switch1/2
  Gas/1 -> Switch1/1
  Constant3/1 -> Switch1/3
  NOTSET1/1 -> Mux/5  "rotv_trg"
  NOTSET2/1 -> Mux/4  "Trq_trg"
  Switch1/1 -> Mux/3  "Load"
  NOTSET0/1 -> Mux/2  "FuelCutOff"
  Switch/1 -> Mux/1  "set_ISC"

== system generic_src/CarMaker/IPG Vehicle/PowerTrain/PTControl Example/PTControl Example/ISG ==
  Key : Inport
  Constant : Constant
  Constant1 : Constant  Value=0
  KeyPos_KeyIn_Starter : Constant  Value=4
  Mux : Mux  Inputs=3
  NOTSET : Constant  Value=-99999
  NOTSET1 : Constant  Value=-99999
  Relational Operator1 : RelationalOperator  Operator===  OutDataTypeStr=boolean  RndMeth=Nearest
  Switch : Switch  Criteria=u2 ~= 0
  ISGOut : Outport  VectorParamsAs1DForOutWhenUnconnected=off
  wires:
  KeyPos_KeyIn_Starter/1 -> Relational Operator1/2
  Constant/1 -> Switch/1
  Constant1/1 -> Switch/3
  Relational Operator1/1 -> Switch/2
  Key/1 -> Relational Operator1/1
  Switch/1 -> Mux/1  "Load"
  NOTSET/1 -> Mux/2  "Trq_trg"
  NOTSET1/1 -> Mux/3  "rotv_trg"
  Mux/1 -> ISGOut/1

== system generic_src/CarMaker/IPG Vehicle/PowerTrain/PTControl Example/PTControl Example/PTC ==
  Key : Inport
  Engine_on : Inport  Port=2
  Constant : Constant
  Constant1 : Constant  Value=0
  Ground : Ground
  KeyPos2OperState : Lookup  InputValues=[0 1 2 3 4 5 6 7 8 9]  Table=[0 1 2 3 3 3 3 3 3 3]
  KeyPos_KeyIn_PowerOn : Constant  Value=3
  Logical Operator : Logic  AllPortsSameDT=off  OutDataTypeStr=boolean
  Mode_EngineDrive : Constant  Value=8
  Mux : Mux
  OperState_Driving : Constant  Value=4
  OperState_PowerOn : Constant  Value=3
  Relational Operator : RelationalOperator  OutDataTypeStr=boolean  RndMeth=Nearest
  Relational Operator1 : RelationalOperator  OutDataTypeStr=boolean  RndMeth=Nearest
  Switch : Switch  Criteria=u2 ~= 0
  Switch1 : Switch  Criteria=u2 ~= 0
  PTC MiscOut : Outport  VectorParamsAs1DForOutWhenUnconnected=off
  wires:
  KeyPos_KeyIn_PowerOn/1 -> Relational Operator/2
  Ground/1 -> Mux/2  "OperationError"
  Mux/1 -> PTC MiscOut/1
  Key/1 -> KeyPos2OperState/1, Relational Operator/1
  Constant/1 -> Switch/1
  Constant1/1 -> Switch/3
  Relational Operator/1 -> Switch/2  "Ignition"
  OperState_Driving/1 -> Switch1/1
  Switch1/1 -> Mux/1  "OperationState"
  KeyPos2OperState/1 -> Relational Operator1/1, Switch1/3  "OperationState"
  Logical Operator/1 -> Switch1/2
  Engine_on/1 -> Logical Operator/1
  Relational Operator1/1 -> Logical Operator/2
  OperState_PowerOn/1 -> Relational Operator1/2
  Switch/1 -> Mux/4  "Ignition"
  Mode_EngineDrive/1 -> Mux/3

== system generic_src/CarMaker/IPG Vehicle/PowerTrain/PTControl Example/PTControl_In/CreateBus PTC BatteryHVIn ==
  In : Inport
  BusCreator : BusCreator  Inputs=8
  Demux : Demux  Outputs=8
      settings: DisplayOption=none
  Out : Outport  VectorParamsAs1DForOutWhenUnconnected=off
  wires:
  Demux/5 -> BusCreator/5  "PTC BattHVIn Energy"
  Demux/4 -> BusCreator/4  "PTC BattHVIn AOC"
  BusCreator/1 -> Out/1
  Demux/2 -> BusCreator/2  "PTC BattHVIn SOH"
  Demux/3 -> BusCreator/3  "PTC BattHVIn Current"
  Demux/1 -> BusCreator/1  "PTC BattHVIn SOC"
  Demux/6 -> BusCreator/6  "PTC BattHVIn Pwr_max"
  Demux/8 -> BusCreator/8  "PTC BattHVIn TempCool_out"
  In/1 -> Demux/1
  Demux/7 -> BusCreator/7  "PTC BattHVIn Temp"
